simulink model "InductionHeating_bb_4"  (R2026b)
settings: Solver=FixedStepDiscrete  StopTime=0.008
PostLoadFcn:
  | Ts = 1e-6;Ts_fpga=10e-9;   R=3; Capa=300e-9;L=100e-6;Pejo_factor=1;
InitFcn:
  | Ts = 1e-6;Ts_fpga=10e-9;   R=3; Capa=300e-9;L=100e-6;Pejo_factor=1;
undefined symbols (not defined in the file or in its folder): DiscIntNeverNeededParam, ee_sli_rtmsupport, gcbh, isSetWhenUndefinedState, MATESOCwDio
libraries: fl_lib x67, nesl_utility x40, hdlsllib x32, simulink x15, eeGeneralControl x9, ee_lib x3
(part 5 of 7)

== system InductionHeating_bb_4/soc16/PWM_Generator at Ts1 ==
  note: must change deadtime because integrator reset must be scalar
  PWMsteps : Inport
  PWMstepsON : Inport  Port=2
  deatime(s) : Inport  Port=3
  enable : Inport  Port=4
  Constant : Constant  Value=[0 0]  OutDataTypeStr=boolean  SampleTime=Ts
  Data Type Conversion1 : DataTypeConversion  Commented=on  OutDataTypeStr=single  RndMeth=Nearest  SaturateOnIntegerOverflow=off
  Discrete-Time Integrator : DiscreteIntegrator  Commented=on  gainval=1  ExternalReset=level  SampleTime=Ts  LimitOutput=on  ICPrevOutput=DiscIntNeverNeededParam  ICPrevScaledInput=DiscIntNeverNeededParam
  Logical Operator1 : Logic  Operator=NOT  AllPortsSameDT=off  OutDataTypeStr=boolean
  Logical Operator2 : Logic  Commented=on  AllPortsSameDT=off  OutDataTypeStr=boolean
  Logical Operator3 : Logic  Commented=on  Operator=NOT  AllPortsSameDT=off  OutDataTypeStr=boolean
  Mux1 : Mux  Inputs=2
  PWM generator : Subsystem
  Relational Operator1 : RelationalOperator  Commented=on  Operator=>  OutDataTypeStr=boolean  RndMeth=Simplest  InputSameDT=off
  Switch : Switch  Criteria=u2 ~= 0  SaturateOnIntegerOverflow=off  InputSameDT=off
  gate : Outport  VectorParamsAs1DForOutWhenUnconnected=off
  wires:
  Constant/1 -> Switch/3
  enable/1 -> Switch/2
  Switch/1 -> gate/1
  PWMstepsON/1 -> PWM generator/2(stepON)
  PWMsteps/1 -> PWM generator/1(steps)
  PWM generator/1(pulse) -> Mux1/1, Logical Operator1/1
  Discrete-Time Integrator/1 -> Relational Operator1/1
  Relational Operator1/1 -> Logical Operator2/1
  Logical Operator3/1 -> Discrete-Time Integrator/2
  Logical Operator1/1 -> Mux1/2
  Mux1/1 -> Logical Operator2/2, Switch/1, Data Type Conversion1/1, Logical Operator3/1
  Data Type Conversion1/1 -> Discrete-Time Integrator/1  "Simulink-PS Converter1"
  deatime(s)/1 -> Relational Operator1/2

== system InductionHeating_bb_4/soc16/PWM_Generator at Ts2 ==
  note: must change deadtime because integrator reset must be scalar
  PWMsteps : Inport
  PWMstepsON : Inport  Port=2
  deatime(s) : Inport  Port=3
  enable : Inport  Port=4
  Constant : Constant  Value=[0 0]  OutDataTypeStr=boolean  SampleTime=Ts
  Data Type Conversion1 : DataTypeConversion  Commented=on  OutDataTypeStr=single  RndMeth=Nearest  SaturateOnIntegerOverflow=off
  Discrete-Time Integrator : DiscreteIntegrator  Commented=on  gainval=1  ExternalReset=level  SampleTime=Ts  LimitOutput=on  ICPrevOutput=DiscIntNeverNeededParam  ICPrevScaledInput=DiscIntNeverNeededParam
  Logical Operator1 : Logic  Operator=NOT  AllPortsSameDT=off  OutDataTypeStr=boolean
  Logical Operator2 : Logic  Commented=on  AllPortsSameDT=off  OutDataTypeStr=boolean
  Logical Operator3 : Logic  Commented=on  Operator=NOT  AllPortsSameDT=off  OutDataTypeStr=boolean
  Mux1 : Mux  Inputs=2
  PWM generator : Subsystem
  Relational Operator1 : RelationalOperator  Commented=on  Operator=>  OutDataTypeStr=boolean  RndMeth=Simplest  InputSameDT=off
  Switch : Switch  Criteria=u2 ~= 0  SaturateOnIntegerOverflow=off  InputSameDT=off
  gate : Outport  VectorParamsAs1DForOutWhenUnconnected=off
  wires:
  deatime(s)/1 -> Relational Operator1/2
  Data Type Conversion1/1 -> Discrete-Time Integrator/1  "Simulink-PS Converter1"
  Mux1/1 -> Logical Operator3/1, Data Type Conversion1/1, Switch/1, Logical Operator2/2
  Logical Operator1/1 -> Mux1/2
  Logical Operator3/1 -> Discrete-Time Integrator/2
  Relational Operator1/1 -> Logical Operator2/1
  Discrete-Time Integrator/1 -> Relational Operator1/1
  PWM generator/1(pulse) -> Logical Operator1/1, Mux1/1
  PWMsteps/1 -> PWM generator/1(steps)
  PWMstepsON/1 -> PWM generator/2(stepON)
  Switch/1 -> gate/1
  enable/1 -> Switch/2
  Constant/1 -> Switch/3

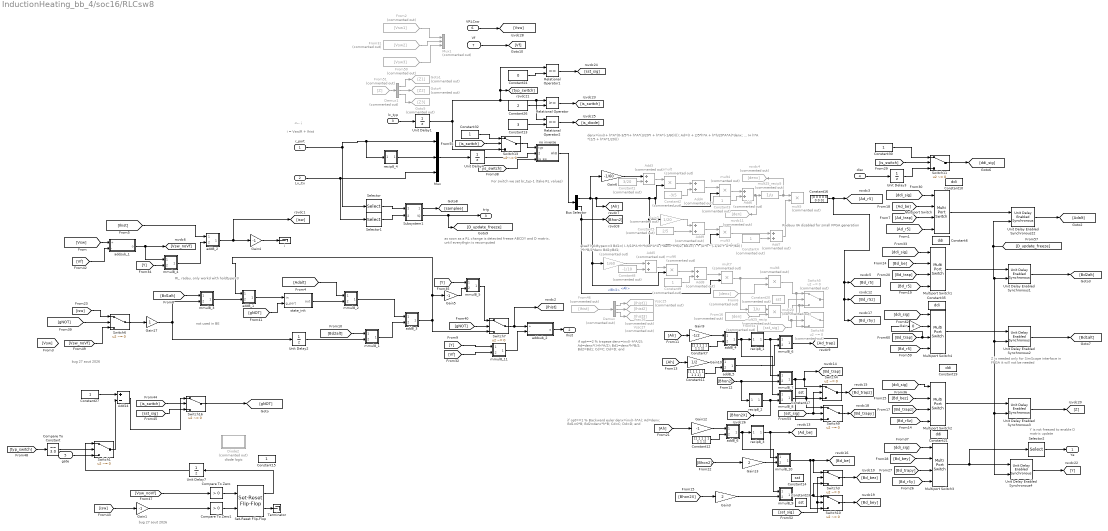
== system InductionHeating_bb_4/soc16/RLCsw8 ==
  note: Radauu IIA disabled for small FPGA generation
  note: bug 27 aout 2026
  note: bug 27 aout 2026
  note: diode logic
  note: Y is not freezed to
      | enable D matrix update
  note: as soon as a RL change is detected
      | freeze ABCDY and D matrix, until everythgin is recomputed
  note: For switch we set br_typ-1 (take RL values)
  note: if opt==1 % Backward euler
      | denx=inv(I-h*A);
      | Ad=denx;
      | Bd1=0*B;
      | Bd2=denx*h*B;
      | Cd=C;
      | Dd=D;
      | end
  note: if opt==2 % trapeze
      | denx=inv(I-h*A/2);
      | Ad=denx*(I+h*A/2);
      | Bd1=denx*h*B/2;
      | Bd2=Bd1;
      | Cd=C;
      | Dd=D;
      | end
  note: RL, radau, only workd with holdtype=3
  note: elseif holdtype==3
      | Bd1=( I-h/10*A+h*h/60*A*A )*denx*h*B/2;
      | Bd1=( I + (A*h * (-1/10 + A*h*/60) ) )*h*B/2*denx
      | Bd2=Bd1;
  note: denx=inv(I+ h*A*(0-3/5*I+ h*A*(3/20*I + h*A*(-1/60))));
      | Ad=(I + 2/5*h*A + h*h/20*A*A)*denx;
      | ... I+ h*A *(2/5 + h*A*1/20)))
  note: <-- i
  note: i = Vsw/R + Ihist
  note: Z is needed only for SimScape interface
      | in FPGA it will not be needed
  note: not used in BE
  r_port : Inport
  Lx_Cx : Inport  Port=2
  lc_typ : Inport  Port=3
  disc : Inport  Port=4
  gate : Inport  Port=5
  VRLCsw : Inport  Port=6
  Vf : Inport  Port=7
  Add14 : Sum  Inputs=+-
  Add{3..9} (7 alike) : Sum  Commented=on  Inputs=2
  Bus Selector : BusSelector  OutputSignals=Ah,Bh/2
  Compare To Constant : simulink/Logic and Bit Operations/Compare To Constant  relop===  const=3.0  OutDataTypeStr=boolean
  Compare To Zero : simulink/Logic and Bit Operations/Compare To Zero  relop=>  OutDataTypeStr=boolean
  Compare To Zero1 : simulink/Logic and Bit Operations/Compare To Zero  relop=>  OutDataTypeStr=boolean
  Constant1 : Constant  Commented=on  Value=3/20  OutDataTypeStr=single  SampleTime=Ts
  Constant{6,10,19,21,35} (5 alike) : Constant  Value=ddi  SampleTime=Ts
  Constant11 : Constant  Value=[1 1 1 1 1 1 1 1]  OutDataTypeStr=single  SampleTime=Ts
  Constant12 : Constant  Value=[1 1 1 1 1 1 1 1]  OutDataTypeStr=single  SampleTime=Ts
  Constant13 : Constant  Value=3  OutDataTypeStr=uint8  SampleTime=Ts
  Constant14 : Constant  Value=sst  SampleTime=Ts
  Constant15 : Constant  OutDataTypeStr=boolean  SampleTime=Ts
  Constant16 : Constant  Value=[0 0 0 0 0 0 0 0]  OutDataTypeStr=single  SampleTime=Ts
  Constant17 : Constant  Value=sst  SampleTime=Ts
  Constant2 : Constant  Commented=on  Value=-3/5  OutDataTypeStr=single  SampleTime=Ts
  Constant20 : Constant  Commented=on  Value=sst  SampleTime=Ts
  Constant23 : Constant  Value=sst  SampleTime=Ts
  Constant24 : Constant  Value=0  OutDataTypeStr=uint8  SampleTime=Ts
  Constant26 : Constant  Value=2  OutDataTypeStr=uint8  SampleTime=Ts
  Constant27 : Constant  OutDataTypeStr=boolean  SampleTime=Ts
  Constant3 : Constant  Commented=on  OutDataTypeStr=single  SampleTime=Ts
  Constant30 : Constant  OutDataTypeStr=uint8  SampleTime=Ts
  Constant32 : Constant  OutDataTypeStr=uint8  SampleTime=Ts
  Constant4 : Constant  Commented=on  OutDataTypeStr=single  SampleTime=Ts
  Constant5 : Constant  Commented=on  Value=2/5  OutDataTypeStr=single  SampleTime=Ts
  Constant7 : Constant  Value=[1 1 1 1 1 1 1 1]  OutDataTypeStr=single  SampleTime=Ts
  Constant8 : Constant  Commented=on  Value=-1/10  OutDataTypeStr=single  SampleTime=Ts
  Constant9 : Constant  Commented=on  OutDataTypeStr=single  SampleTime=Ts
  Demux : Demux  Commented=on  Outputs=3
  Demux1 : Demux  Commented=on  Outputs=3
  Diode2 : Subsystem  Commented=on  AncestorBlock=simetranss/FPGA/Diode  mask(MATE Diode (Pejovic-based)){VF=0.8, RON=1e-1, LON=1e-6*Pejo_factor, TS=Ts}
      mask prompts: VF "Threshold voltage (V)"; RON "Conduction resistance (Ohms)"; LON "Pejovic Equivalent Inductance during conduction (H)"; TS "Sample time (s)"
      mask help:
      | Implements a diode using a Pejovic switch model.
      |
      | Diode turns ON when Vdiode> Vthreshold and turns OFF when current is 0.
      |
      | The model is based on a Pejovic switch, with equivalent inductance during conduction Lon equal to Lon/Ts=Ts/Coff
      | where Ts is the sample time in second and Coff is the equivalent capacitance when the diode in not conducting.
  From16 : From  Commented=on  GotoTag=den
  From2 : From  Commented=on  GotoTag=Vsw1
  From31 : From  Commented=on  GotoTag=Vsw2
  From46 : From  Commented=on  GotoTag=Ihist
  From50 : From  Commented=on  GotoTag=Vsw3
  From51 : From  Commented=on  GotoTag=Z
  From54 : From  Commented=on  GotoTag=sst_sig
  From6 : From  Commented=on  GotoTag=denx
  Gain : Gain  Gain=0
  Gain{1,4..5,12} (4 alike) : Gain  Gain=-1
  Gain10 : Gain  Gain=1/2
  Gain13 : Gain  Gain=2
  Gain17 : Gain
  Gain3 : Gain  Gain=2
  Gain6 : Gain  Gain=-1/60
  Gain7 : Gain  Commented=on  Gain=1/20
  Gain8 : Gain  Commented=on  Gain=1/60
  Gain9 : Gain  Gain=-1/2
  Goto1 : Goto  Commented=on  GotoTag=Z1
  Goto4 : Goto  Commented=on  GotoTag=Z2
  Goto5 : Goto  Commented=on  GotoTag=Z3
  Multiport Switch{,1..4} (5 alike) : MultiPortSwitch  SaturateOnIntegerOverflow=off  InputSameDT=off
  Mux : Mux  Inputs=3
  Mux1 : Mux  Commented=on  Inputs=3
  Relational Operator : RelationalOperator  OutDataTypeStr=boolean  RndMeth=Simplest  InputSameDT=off
  Relational Operator1 : RelationalOperator  Operator===  OutDataTypeStr=boolean  RndMeth=Simplest  InputSameDT=off
  Relational Operator2 : RelationalOperator  Operator===  OutDataTypeStr=boolean  RndMeth=Simplest  InputSameDT=off
  Selector : Selector  InputPortWidth=8  IndexOptions=Index vector (dialog)  Indices=1  OutputSizes=1  RuntimeRangeChecks=off
  Selector1 : Selector  InputPortWidth=8  IndexOptions=Index vector (dialog)  Indices=1  OutputSizes=1  RuntimeRangeChecks=off
  Selector2 : Selector  InputPortWidth=8  IndexOptions=Index vector (dialog)  Indices=[1]  OutputSizes=1  RuntimeRangeChecks=off
  Set-Reset Flip-Flop : eeGeneralControl/Set-Reset Flip-Flop  LabelModeActiveChoice=Discrete  UndefState=Set  Q0=0  Ts=Ts
  Subsystem1 : Subsystem
  Switch1 : Switch  Criteria=u2 ~= 0  Threshold=0.5  SaturateOnIntegerOverflow=off  InputSameDT=off
  Switch{3..4,6..7,9..11} (7 alike) : Switch  Criteria=u2 ~= 0  SaturateOnIntegerOverflow=off  InputSameDT=off
  Switch13 : Switch  Criteria=u2 ~= 0  OutDataTypeStr=uint8  SaturateOnIntegerOverflow=off  InputSameDT=off
  Switch16 : Switch  Criteria=u2 ~= 0  Threshold=0.5  SaturateOnIntegerOverflow=off  InputSameDT=off
  Switch5 : Switch  Commented=on  Criteria=u2 ~= 0  SaturateOnIntegerOverflow=off  InputSameDT=off
  Switch8 : Switch  Commented=on  Criteria=u2 ~= 0  SaturateOnIntegerOverflow=off  InputSameDT=off
  Terminator : Terminator
  Unit Delay Enabled Synchronous{1..4,22} (5 alike) : hdlsllib/Discrete/Unit Delay Enabled Synchronous  InitialCondition=0.0  SampleTime=-1
  Unit Delay1 : UnitDelay  InitialCondition=1  SampleTime=Ts
  Unit Delay2 : UnitDelay  SampleTime=-1
  Unit Delay3 : UnitDelay  InitialCondition=1  SampleTime=Ts
  Unit Delay4 : UnitDelay  InitialCondition=1  SampleTime=Ts
  Unit Delay7 : UnitDelay  SampleTime=Ts
  Vssc25 : Goto  Commented=on  GotoTag=Ihist1
  Vssc26 : Goto  Commented=on  GotoTag=Ihist2
  Vssc27 : Goto  Commented=on  GotoTag=Ihist3
  add8_1 : Subsystem
      mask Display: disp('add8')
  add8_2 : Subsystem
      mask Display: disp('add8')
  add8_3 : Subsystem
      mask Display: disp('add8')
  add8_4 : Subsystem
      mask Display: disp('add8')
  add8_5 : Subsystem
      mask Display: disp('add8')
  add8_6 : Subsystem
      mask Display: disp('add8')
  addsub_1 : Subsystem
      mask Display: disp('addsub8')
  addsub_2 : Subsystem
      mask Display: disp('addsub8')
  i : Terminator
  mmul8_1 : Subsystem
      mask Display: disp('X8')
  mmul8_10 : Subsystem
      mask Display: disp('X8')
  mmul8_11 : Subsystem
      mask Display: disp('X8')
  mmul8_2 : Subsystem
      mask Display: disp('X8')
  mmul8_3 : Subsystem
      mask Display: disp('X8')
  mmul8_4 : Subsystem
      mask Display: disp('X8')
  mmul8_5 : Subsystem
      mask Display: disp('X8')
  mmul8_6 : Subsystem
      mask Display: disp('X8')
  mmul8_7 : Subsystem
      mask Display: disp('X8')
  mmul8_8 : Subsystem
      mask Display: disp('X8')
  mmul8_9 : Subsystem
      mask Display: disp('X8')
  mult{,3..8,20} (8 alike) : Product  Commented=on
  mult25_recip : Math  Commented=on  Operator=reciprocal
  mult25_recip5 : Math  Commented=on  Operator=reciprocal
  no inverse : Subsystem
  recip8_1 : Subsystem
      mask help: This block is to allow SharingFactor=8 in FPGA
      mask Display: disp('inv8')
  recip8_2 : Subsystem
      mask help: This block is to allow SharingFactor=8 in FPGA
      mask Display: disp('inv8')
  recip8_3 : Subsystem
      mask help: This block is to allow SharingFactor=8 in FPGA
      mask Display: disp('inv8')
  recip8_4 : Subsystem
      mask help: This block is to allow SharingFactor=8 in FPGA
      mask Display: disp('inv8')
  rsvdc11 : Goto  Commented=on  GotoTag=den
  rsvdc4 : Goto  Commented=on  GotoTag=denx
  state_init : Subsystem
  Ye : Outport
  Ihist : Outport  Port=2
  trig : Outport  Port=3
  wires:
  Switch16/1 -> [gNOT]
  Add14/1 -> Switch16/1
  [gNOT] -> state_init/2(g_port)
  state_init/1(out) -> mmul8_2/2(In2)
  [gNOT] -> Switch7/2
  [gNOT] -> Switch6/2
  Constant27/1 -> Add14/1
  Gain17/1 -> mmul8_3/2(In2), Unit Delay2/1
  Gain5/1 -> mmul8_5/2(In2)
  [Y] -> mmul8_5/1(In1)
  mmul8_5/1(Out1) -> Switch7/1
  mmul8_4/1(Out1) -> add8_2/2(In2)
  [Y] -> mmul8_4/2(In2)
  Switch10/1 -> [Bd_bey]
  mmul8_7/1(Out1) -> Switch4/1, [Bd_trap], Switch9/3
  mmul8_8/1(Out1) -> Switch4/3, Switch9/1
  Switch9/1 -> [Bd_trapy]
  [Bd_r5y] -> Multiport Switch3/4
  [Bd_trapy] -> Multiport Switch3/3
  [Bd_bey] -> Multiport Switch3/2
  Switch4/1 -> [Bd_trapz]
  mult8/1 -> Switch5/1, Switch8/3
  [Bd_bez] -> Multiport Switch2/2
  [Bd_trapz] -> Multiport Switch2/3
  [Bd_r5z] -> Multiport Switch2/4
  mmul8_2/1(Out1) -> add8_3/1(In1)
  [isw] -> Switch6/1
  Switch6/1 -> Gain17/1
  add8_2/1(Out1) -> [isw], Gain4/1
  [Ihist] -> add8_2/1(In1)
  Gain4/1 -> i/1
  add8_1/1(Out1) -> state_init/1(in)
  add8_3/1(Out1) -> add8_1/1(In1), Gain5/1, Switch7/3
  Gain6/1 -> Add3/1
  Constant1/1 -> Add3/2
  mult/1 -> Add4/1
  Add3/1 -> mult/1
  Constant2/1 -> Add4/2
  Add4/1 -> mult4/1
  mult4/1 -> Add6/1
  Constant3/1 -> Add6/2
  Add6/1 -> rsvdc11/1, mult25_recip5/1
  Constant4/1 -> Add7/2
  Constant5/1 -> Add9/2
  Add9/1 -> mult3/1
  Gain7/1 -> Add9/1
  mult3/1 -> Add7/1
  Add7/1 -> mult5/2
  [Adalt] -> mmul8_2/1(In1)
  mult25_recip5/1 -> rsvdc4/1, mult5/1
  Constant9/1 -> Add8/2
  Add5/1 -> mult6/1
  mult6/1 -> Add8/1
  Constant8/1 -> Add5/2
  Gain8/1 -> Add5/1
  Add8/1 -> mult7/1
  mult7/1 -> mult25_recip/1, mult8/1
  From6/1 -> mult8/2
  Bus Selector/1 -> Gain6/1, [Ah], mult3/2, Gain7/1, mult4/2, mult/2, Gain8/1, mult6/2  "<Ah>"
  Bus Selector/2 -> mult7/2, [Bhon2]  "<Bh/2>"
  [Ah] -> Gain9/1
  Gain9/1 -> add8_4/1(In1)
  Constant7/1 -> add8_4/2(In2)
  add8_4/1(Out1) -> recip8_1/1(In1), mmul8_8/1(In1)
  add8_5/1(Out1) -> mmul8_6/2(In2)
  Constant11/1 -> add8_5/2(In2)
  Gain10/1 -> add8_5/1(In1)
  [Ah] -> Gain10/1
  recip8_1/1(Out1) -> mmul8_7/1(In1), mmul8_6/1(In1)
  [Bhon2] -> recip8_2/1(In1), mmul8_7/2(In2)
  mmul8_6/1(Out1) -> [Ad_trap]
  mmul8_3/1(Out1) -> add8_1/2(In2)
  recip8_3/1(Out1) -> mmul8_10/1(In1), [Ad_be]
  [Bhon2] -> Gain13/1
  add8_6/1(Out1) -> recip8_3/1(In1), mmul8_9/1(In1)
  Constant12/1 -> add8_6/2(In2)
  Gain12/1 -> add8_6/1(In1)
  [Ah] -> Gain12/1
  Gain13/1 -> mmul8_10/2(In2)
  [Ad_r5] -> Multiport Switch/4
  [Ad_trap] -> Multiport Switch/3
  [Ad_be] -> Multiport Switch/2
  [Bd_r5] -> Multiport Switch1/4
  [Bd_trap] -> Multiport Switch1/3
  [Bd_be] -> Multiport Switch1/2
  recip8_2/1(Out1) -> [Bhon2X], mmul8_8/2(In2)
  Gain3/1 -> mmul8_9/2(In2)
  mmul8_9/1(Out1) -> Switch3/3, Switch10/1
  mmul8_10/1(Out1) -> Switch3/1, [Bd_be], Switch10/3
  Switch3/1 -> [Bd_bez]
  From16/1 -> mult20/2
  mult25_recip/1 -> mult20/1
  mult20/1 -> Switch5/3, Switch8/1
  Mux/1 -> Unit Delay4/1
  lc_typ/1 -> Unit Delay1/1
  no inverse/1(AhB) -> Bus Selector/1
  Constant26/1 -> Relational Operator/2
  Relational Operator/1 -> [is_switch]
  [is_switch] -> Switch16/2
  Constant24/1 -> Relational Operator1/2
  Relational Operator1/1 -> [sst_sig]
  [sst_sig] -> Switch16/3
  From46/1 -> Demux/1
  Demux/1 -> Vssc25/1
  Demux/2 -> Vssc26/1
  Demux/3 -> Vssc27/1
  From31/1 -> Mux1/2
  From2/1 -> Mux1/1
  From50/1 -> Mux1/3
  From51/1 -> Demux1/1
  Demux1/2 -> Goto4/1
  Demux1/1 -> Goto1/1
  Demux1/3 -> Goto5/1
  [is_switch] -> Switch11/2
  disc/1 -> Unit Delay3/1
  Constant30/1 -> Switch11/1
  Switch11/1 -> [ddi_sig]
  [ddi_sig] -> Multiport Switch/1
  [ddi_sig] -> Multiport Switch1/1
  [ddi_sig] -> Multiport Switch2/1
  [ddi_sig] -> Multiport Switch3/1
  [sst_sig] -> Switch3/2, Switch10/2
  [sst_sig] -> Switch4/2, Switch9/2
  From54/1 -> Switch8/2, Switch5/2
  r_port/1 -> recip8_4/1(In1), Mux/1, Selector/1
  ? -> ?
  Switch13/1 -> no inverse/1(typ)
  Constant32/1 -> Switch13/1
  mmul8_1/1(Out1) -> add8_3/2(In2)
  Unit Delay2/1 -> mmul8_1/2(In2)
  [ddi_sig] -> Multiport Switch4/1
  [Bd_r5] -> Multiport Switch4/4
  [Bd_trap] -> Gain/1, Multiport Switch4/3
  Lx_Cx/1 -> Mux/3, Selector1/1
  [Bd2alt] -> mmul8_1/1(In1)
  [Bd1alt] -> mmul8_3/1(In1)
  VRLCsw/1 -> [Vsw]
  Multiport Switch1/1 -> Unit Delay Enabled Synchronous1/1
  Unit Delay Enabled Synchronous22/1 -> [Adalt]
  Multiport Switch/1 -> Unit Delay Enabled Synchronous22/1
  Unit Delay Enabled Synchronous1/1 -> [Bd2alt]
  Multiport Switch4/1 -> Unit Delay Enabled Synchronous2/1
  Unit Delay Enabled Synchronous2/1 -> [Bd1alt]
  Multiport Switch2/1 -> Unit Delay Enabled Synchronous3/1
  Unit Delay Enabled Synchronous3/1 -> [Z]
  Multiport Switch3/1 -> Unit Delay Enabled Synchronous4/1, Selector2/1
  Unit Delay Enabled Synchronous4/1 -> [Y]
  Subsystem1/1(q_port) -> [samplee]
  Selector/1 -> Subsystem1/1(trig)
  Selector1/1 -> Subsystem1/2(trig1)
  Subsystem1/2(!Q) -> [D_update_freeze], trig/1
  [D_update_freeze] -> Unit Delay Enabled Synchronous22/2, Unit Delay Enabled Synchronous2/2, Unit Delay Enabled Synchronous4/2, Unit Delay Enabled Synchronous3/2, Unit Delay Enabled Synchronous1/2
  Selector2/1 -> Ye/1
  Gain/1 -> Multiport Switch4/2
  [is_switch] -> Switch13/2
  Unit Delay4/1 -> no inverse/2(R_Rx_Lx_Cx)
  Unit Delay1/1 -> Relational Operator2/1, Relational Operator/1, Relational Operator1/1, [typ_switch], Switch13/3
  Unit Delay3/1 -> Switch11/3
  Switch7/1 -> [Ihist], addsub_2/1(+)
  addsub_2/1(o) -> Ihist/1
  [Y] -> mmul8_11/1(In1)
  mmul8_11/1(Out1) -> addsub_2/2(-)
  [Vsw] -> addsub_1/1(+)
  addsub_1/1(o) -> mmul8_4/1(In1), [Vsw_noVf]
  [Vf] -> mmul8_11/2(In2)
  Vf/1 -> [Vf]
  [Vf] -> addsub_1/2(-)
  Set-Reset Flip-Flop/2 -> Terminator/1
  [isw] -> Gain1/1
  Compare To Zero/1 -> Set-Reset Flip-Flop/1
  [Vsw_noVf] -> Compare To Zero/1
  Compare To Zero1/1 -> Set-Reset Flip-Flop/2
  Unit Delay7/1 -> Switch1/1
  [typ_switch] -> Compare To Constant/1
  gate/1 -> Switch1/3
  Switch1/1 -> Add14/2
  Compare To Constant/1 -> Switch1/2
  Constant13/1 -> Relational Operator2/2
  Relational Operator2/1 -> [is_diode]
  recip8_4/1(Out1) -> Mux/2
  [is_switch] -> no inverse/3(is_sw)
  Gain1/1 -> Compare To Zero1/1
  [Vsw_noVf] -> Switch6/3
  Set-Reset Flip-Flop/1 -> Unit Delay7/1
  Constant16/1 -> [Bd_r5y], [Bd_r5z], [Bd_r5], [Ad_r5]
  [Bhon2X] -> Gain3/1

== system InductionHeating_bb_4/MATEwDiode/C1/RC.1 ==
  RLC : Inport
  typ : Inport  Port=2
  Bus Creator : BusCreator  Inputs=2
  Demux : Demux  Outputs=2
  Divide : Product  Inputs=*/
  Divide1 : Product  Inputs=/
  Divide3 : Product
  Divide4 : Product  Inputs=/
  Divide5 : Product  Inputs=/
  Gain : Gain  Gain=-Ts
  Gain1 : Gain  Gain=Ts/2
  Gain2 : Gain  Gain=Ts/2
  Gain3 : Gain  Gain=-Ts
  Switch : Switch  Criteria=u2 > Threshold  SaturateOnIntegerOverflow=off  InputSameDT=off
  Switch1 : Switch  Criteria=u2 > Threshold  SaturateOnIntegerOverflow=off  InputSameDT=off
  AhB : Outport
  wires:
  Gain2/1 -> Switch1/1  "Bh/2"
  Gain3/1 -> Switch/1  "Ah"
  Gain1/1 -> Switch1/3  "Bh/2"
  Gain/1 -> Switch/3  "Ah"
  typ/1 -> Switch/2, Switch1/2
  Switch1/1 -> Bus Creator/2  "Bh/2"
  Switch/1 -> Bus Creator/1  "Ah"
  Divide3/1 -> Gain3/1
  Divide4/1 -> Divide3/2, Gain2/1
  RLC/1 -> Demux/1
  Bus Creator/1 -> AhB/1
  Demux/1 -> Divide5/1, Divide/1
  Divide1/1 -> Gain1/1
  Divide/1 -> Gain/1
  Demux/2 -> Divide1/1, Divide/2, Divide4/1
  Divide5/1 -> Divide3/1

== system InductionHeating_bb_4/MATEwDiode/C1/Rsw ==
  Variable Resistor : fl_lib/Electrical/Electrical Elements/Variable Resistor  Rmin=1e-8 Ohm  thermalEnable=false  thermal_mass=1 J/K  i_specify=off  i_priority=None  i=0 A  i_nominal_specify=off  i_nominal_value=1  i_nominal_unit=A  v_specify=off  v_priority=None  v=0 V  v_nominal_specify=off  v_nominal_value=1  v_nominal_unit=V  T_specify=off  T_priority=None  T=300 K  T_nominal_specify=off  T_nominal_value=1  T_nominal_unit=K
  + : PMIOPort  Side=Left
  R : PMIOPort  Port=2  Side=Left
  - : PMIOPort  Port=3  Side=Right
  connections:
  Variable Resistor/RConn1 -- -/RConn1
  Variable Resistor/LConn2 -- +/RConn1
  R/RConn1 -- Variable Resistor/LConn1

== system InductionHeating_bb_4/MATEwDiode/C1/state_init ==
  in : Inport
  g : Inport  Port=2
  Gain18 : Gain
  Relational Operator1 : RelationalOperator  Operator=~=  OutDataTypeStr=boolean  RndMeth=Simplest  InputSameDT=off
  Switch16 : Switch  Criteria=u2 ~= 0  Threshold=0.5  SaturateOnIntegerOverflow=off  InputSameDT=off
  Unit Delay6 : UnitDelay  SampleTime=-1
  Unit Delay7 : UnitDelay  SampleTime=Ts
  Unit Delay8 : UnitDelay  SampleTime=Ts
  init_in : Constant  Value=0
  out : Outport
  wires:
  Unit Delay8/1 -> Relational Operator1/1
  Relational Operator1/1 -> Gain18/1
  Unit Delay6/1 -> Switch16/3
  init_in/1 -> Unit Delay7/1
  Gain18/1 -> Switch16/2
  Unit Delay7/1 -> Switch16/1
  in/1 -> Unit Delay6/1
  Switch16/1 -> out/1
  g/1 -> Unit Delay8/1, Relational Operator1/2

== system InductionHeating_bb_4/MATEwDiode/C2/RC.1 ==
  RLC : Inport
  typ : Inport  Port=2
  Bus Creator : BusCreator  Inputs=2
  Demux : Demux  Outputs=2
  Divide : Product  Inputs=*/
  Divide1 : Product  Inputs=/
  Divide3 : Product
  Divide4 : Product  Inputs=/
  Divide5 : Product  Inputs=/
  Gain : Gain  Gain=-Ts
  Gain1 : Gain  Gain=Ts/2
  Gain2 : Gain  Gain=Ts/2
  Gain3 : Gain  Gain=-Ts
  Switch : Switch  Criteria=u2 > Threshold  SaturateOnIntegerOverflow=off  InputSameDT=off
  Switch1 : Switch  Criteria=u2 > Threshold  SaturateOnIntegerOverflow=off  InputSameDT=off
  AhB : Outport
  wires:
  Gain2/1 -> Switch1/1  "Bh/2"
  Gain3/1 -> Switch/1  "Ah"
  Gain1/1 -> Switch1/3  "Bh/2"
  Gain/1 -> Switch/3  "Ah"
  typ/1 -> Switch/2, Switch1/2
  Switch1/1 -> Bus Creator/2  "Bh/2"
  Switch/1 -> Bus Creator/1  "Ah"
  Divide3/1 -> Gain3/1
  Divide4/1 -> Divide3/2, Gain2/1
  RLC/1 -> Demux/1
  Bus Creator/1 -> AhB/1
  Demux/1 -> Divide5/1, Divide/1
  Divide1/1 -> Gain1/1
  Divide/1 -> Gain/1
  Demux/2 -> Divide1/1, Divide/2, Divide4/1
  Divide5/1 -> Divide3/1

== system InductionHeating_bb_4/MATEwDiode/C2/Rsw ==
  Variable Resistor : fl_lib/Electrical/Electrical Elements/Variable Resistor  Rmin=1e-8 Ohm  thermalEnable=false  thermal_mass=1 J/K  i_specify=off  i_priority=None  i=0 A  i_nominal_specify=off  i_nominal_value=1  i_nominal_unit=A  v_specify=off  v_priority=None  v=0 V  v_nominal_specify=off  v_nominal_value=1  v_nominal_unit=V  T_specify=off  T_priority=None  T=300 K  T_nominal_specify=off  T_nominal_value=1  T_nominal_unit=K
  + : PMIOPort  Side=Left
  R : PMIOPort  Port=2  Side=Left
  - : PMIOPort  Port=3  Side=Right
  connections:
  Variable Resistor/RConn1 -- -/RConn1
  Variable Resistor/LConn2 -- +/RConn1
  R/RConn1 -- Variable Resistor/LConn1

== system InductionHeating_bb_4/MATEwDiode/C2/state_init ==
  in : Inport
  g : Inport  Port=2
  Gain18 : Gain
  Relational Operator1 : RelationalOperator  Operator=~=  OutDataTypeStr=boolean  RndMeth=Simplest  InputSameDT=off
  Switch16 : Switch  Criteria=u2 ~= 0  Threshold=0.5  SaturateOnIntegerOverflow=off  InputSameDT=off
  Unit Delay6 : UnitDelay  SampleTime=-1
  Unit Delay7 : UnitDelay  SampleTime=Ts
  Unit Delay8 : UnitDelay  SampleTime=Ts
  init_in : Constant  Value=0
  out : Outport
  wires:
  Unit Delay8/1 -> Relational Operator1/1
  Relational Operator1/1 -> Gain18/1
  Unit Delay6/1 -> Switch16/3
  init_in/1 -> Unit Delay7/1
  Gain18/1 -> Switch16/2
  Unit Delay7/1 -> Switch16/1
  in/1 -> Unit Delay6/1
  Switch16/1 -> out/1
  g/1 -> Unit Delay8/1, Relational Operator1/2

== system InductionHeating_bb_4/MATEwDiode/Cdc/RC.1 ==
  RLC : Inport
  typ : Inport  Port=2
  Bus Creator : BusCreator  Inputs=2
  Demux : Demux  Outputs=2
  Divide : Product  Inputs=*/
  Divide1 : Product  Inputs=/
  Divide3 : Product
  Divide4 : Product  Inputs=/
  Divide5 : Product  Inputs=/
  Gain : Gain  Gain=-Ts
  Gain1 : Gain  Gain=Ts/2
  Gain2 : Gain  Gain=Ts/2
  Gain3 : Gain  Gain=-Ts
  Switch : Switch  Criteria=u2 > Threshold  SaturateOnIntegerOverflow=off  InputSameDT=off
  Switch1 : Switch  Criteria=u2 > Threshold  SaturateOnIntegerOverflow=off  InputSameDT=off
  AhB : Outport
  wires:
  Divide5/1 -> Divide3/1
  Demux/2 -> Divide4/1, Divide/2, Divide1/1
  Divide/1 -> Gain/1
  Divide1/1 -> Gain1/1
  Demux/1 -> Divide/1, Divide5/1
  Bus Creator/1 -> AhB/1
  RLC/1 -> Demux/1
  Divide4/1 -> Gain2/1, Divide3/2
  Divide3/1 -> Gain3/1
  Switch/1 -> Bus Creator/1  "Ah"
  Switch1/1 -> Bus Creator/2  "Bh/2"
  typ/1 -> Switch1/2, Switch/2
  Gain/1 -> Switch/3  "Ah"
  Gain1/1 -> Switch1/3  "Bh/2"
  Gain3/1 -> Switch/1  "Ah"
  Gain2/1 -> Switch1/1  "Bh/2"

== system InductionHeating_bb_4/MATEwDiode/Cdc/Rsw ==
  Variable Resistor : fl_lib/Electrical/Electrical Elements/Variable Resistor  Rmin=1e-8 Ohm  thermalEnable=false  thermal_mass=1 J/K  i_specify=off  i_priority=None  i=0 A  i_nominal_specify=off  i_nominal_value=1  i_nominal_unit=A  v_specify=off  v_priority=None  v=0 V  v_nominal_specify=off  v_nominal_value=1  v_nominal_unit=V  T_specify=off  T_priority=None  T=300 K  T_nominal_specify=off  T_nominal_value=1  T_nominal_unit=K
  + : PMIOPort  Side=Left
  R : PMIOPort  Port=2  Side=Left
  - : PMIOPort  Port=3  Side=Right
  connections:
  R/RConn1 -- Variable Resistor/LConn1
  Variable Resistor/LConn2 -- +/RConn1
  Variable Resistor/RConn1 -- -/RConn1

== system InductionHeating_bb_4/MATEwDiode/Cdc/state_init ==
  in : Inport
  g : Inport  Port=2
  Gain18 : Gain
  Relational Operator1 : RelationalOperator  Operator=~=  OutDataTypeStr=boolean  RndMeth=Simplest  InputSameDT=off
  Switch16 : Switch  Criteria=u2 ~= 0  Threshold=0.5  SaturateOnIntegerOverflow=off  InputSameDT=off
  Unit Delay6 : UnitDelay  SampleTime=-1
  Unit Delay7 : UnitDelay  SampleTime=Ts
  Unit Delay8 : UnitDelay  SampleTime=Ts
  init_in : Constant  Value=0
  out : Outport
  wires:
  g/1 -> Relational Operator1/2, Unit Delay8/1
  Switch16/1 -> out/1
  in/1 -> Unit Delay6/1
  Unit Delay7/1 -> Switch16/1
  Gain18/1 -> Switch16/2
  init_in/1 -> Unit Delay7/1
  Unit Delay6/1 -> Switch16/3
  Relational Operator1/1 -> Gain18/1
  Unit Delay8/1 -> Relational Operator1/1

== system InductionHeating_bb_4/MATEwDiode/Diode1/Pejovic L-C-switch component ==
  gate : Inport
  Vf : Inport  Port=2
  Add : Sum  Inputs=+-
  Add1 : Sum  Inputs=2
  Add2 : Sum  Inputs=+-
  Add3 : Sum  Inputs=2
  Add4 : Sum  Inputs=+-
  CCS1 : fl_lib/Electrical/Electrical Sources/Controlled Current Source
  Gain1 : Gain  Gain=-1/Rsw
  Gain2 : Gain  Gain=Xcomp
  Gain3 : Gain  Gain=-1
  Gain4 : Gain  Gain=-1
  Gain5 : Gain  Gain=1/Rsw*traprule
  Gain6 : Gain  Gain=traprule
  Gain7 : Gain  Gain=-1/Rsw
  PS-Simulink Converter2 : nesl_utility/PS-Simulink Converter  PhysicalDomain=network_engine_domain  SubClassName=ps_output  LeftPortType=input  RightPortType=output  PseudoPeriodic=off  Frequencies=[]  VectorFormat=inherit  Unit=inherit  AffineConversion=off
  Relational Operator1 : RelationalOperator  Operator=~=  OutDataTypeStr=boolean  RndMeth=Simplest  InputSameDT=off
  Resistor : fl_lib/Electrical/Electrical Elements/Resistor  R=Rsw Ohm  i_specify=off  i_priority=None  i=0 A  i_nominal_specify=off  i_nominal_value=1  i_nominal_unit=A  v_specify=off  v_priority=None  v=0 V  v_nominal_specify=off  v_nominal_value=1  v_nominal_unit=V
  Simulink-PS Converter1 : nesl_utility/Simulink-PS Converter  PhysicalDomain=network_engine_domain  SubClassName=ps_input  LeftPortType=input  RightPortType=output  PseudoPeriodic=off  Frequencies=[]  NoiseDistribution=none  NoiseParameters=[]  Unit=1  AffineConversion=off  FilteringAndDerivatives=provide  SimscapeFilterOrder=1  InputFilterTimeConstant=0.001  UdotUserProvided=0
  Switch : Switch  Criteria=u2 > Threshold  Threshold=0.5  SaturateOnIntegerOverflow=off  InputSameDT=off
  Switch4 : Switch  Criteria=u2 > Threshold  Threshold=0.5  SaturateOnIntegerOverflow=off  InputSameDT=off
  Switch5 : Switch  Criteria=u2 ~= 0  Threshold=0.5  SaturateOnIntegerOverflow=off  InputSameDT=off
  Unit Delay1 : UnitDelay  SampleTime=-1
  Unit Delay2 : UnitDelay  SampleTime=Ts
  Unit Delay6 : UnitDelay  SampleTime=Ts
  VS1 : fl_lib/Electrical/Electrical Sensors/Voltage Sensor
  init_in : Constant
  init_out : Terminator
  +V : PMIOPort  Side=Left
  -V : PMIOPort  Port=2  Side=Right
  v : Outport
  i : Outport  Port=2
  wires:
  Add4/1 -> [Vsw], v/1
  Add3/1 -> Simulink-PS Converter1/1
  Gain7/1 -> Add3/2
  [Ihist] -> Add3/1
  Vf/1 -> Gain7/1, Add4/2
  Gain6/1 -> Add2/2
  Add2/1 -> Switch/3
  Gain5/1 -> Add1/2
  [Vsw] -> Gain5/1
  Add1/1 -> Switch/1
  Gain4/1 -> i/1
  Switch5/1 -> [Ihist]
  init_in/1 -> Unit Delay2/1
  Relational Operator1/1 -> Gain2/1
  gate/1 -> Switch/2, Relational Operator1/2, Unit Delay6/1, Switch4/2
  Unit Delay6/1 -> Relational Operator1/1
  Gain2/1 -> Switch5/2
  Gain3/1 -> Switch4/1
  Switch4/1 -> init_out/1
  Unit Delay1/1 -> Switch5/3
  Gain1/1 -> Add/2, Add2/1
  [Ihist] -> Add/1
  PS-Simulink Converter2/1 -> Add4/1
  [Vsw] -> Gain1/1
  Switch/1 -> Unit Delay1/1
  Add/1 -> Gain4/1, Add1/1, Gain6/1
  [Ihist] -> Switch4/3, Gain3/1
  Unit Delay2/1 -> Switch5/1
  connections:
  Resistor/RConn1 -- CCS1/LConn1 -- VS1/RConn2 -- -V/RConn1
  PS-Simulink Converter2/LConn1 -- VS1/RConn1
  CCS1/RConn1 -- Simulink-PS Converter1/RConn1
  Resistor/LConn1 -- VS1/LConn1 -- +V/RConn1 -- CCS1/RConn2

== system InductionHeating_bb_4/MATEwDiode/Diode2/Pejovic L-C-switch component ==
  gate : Inport
  Vf : Inport  Port=2
  Add : Sum  Inputs=+-
  Add1 : Sum  Inputs=2
  Add2 : Sum  Inputs=+-
  Add3 : Sum  Inputs=2
  Add4 : Sum  Inputs=+-
  CCS1 : fl_lib/Electrical/Electrical Sources/Controlled Current Source
  Gain1 : Gain  Gain=-1/Rsw
  Gain2 : Gain  Gain=Xcomp
  Gain3 : Gain  Gain=-1
  Gain4 : Gain  Gain=-1
  Gain5 : Gain  Gain=1/Rsw*traprule
  Gain6 : Gain  Gain=traprule
  Gain7 : Gain  Gain=-1/Rsw
  PS-Simulink Converter2 : nesl_utility/PS-Simulink Converter  PhysicalDomain=network_engine_domain  SubClassName=ps_output  LeftPortType=input  RightPortType=output  PseudoPeriodic=off  Frequencies=[]  VectorFormat=inherit  Unit=inherit  AffineConversion=off
  Relational Operator1 : RelationalOperator  Operator=~=  OutDataTypeStr=boolean  RndMeth=Simplest  InputSameDT=off
  Resistor : fl_lib/Electrical/Electrical Elements/Resistor  R=Rsw Ohm  i_specify=off  i_priority=None  i=0 A  i_nominal_specify=off  i_nominal_value=1  i_nominal_unit=A  v_specify=off  v_priority=None  v=0 V  v_nominal_specify=off  v_nominal_value=1  v_nominal_unit=V
  Simulink-PS Converter1 : nesl_utility/Simulink-PS Converter  PhysicalDomain=network_engine_domain  SubClassName=ps_input  LeftPortType=input  RightPortType=output  PseudoPeriodic=off  Frequencies=[]  NoiseDistribution=none  NoiseParameters=[]  Unit=1  AffineConversion=off  FilteringAndDerivatives=provide  SimscapeFilterOrder=1  InputFilterTimeConstant=0.001  UdotUserProvided=0
  Switch : Switch  Criteria=u2 > Threshold  Threshold=0.5  SaturateOnIntegerOverflow=off  InputSameDT=off
  Switch4 : Switch  Criteria=u2 > Threshold  Threshold=0.5  SaturateOnIntegerOverflow=off  InputSameDT=off
  Switch5 : Switch  Criteria=u2 ~= 0  Threshold=0.5  SaturateOnIntegerOverflow=off  InputSameDT=off
  Unit Delay1 : UnitDelay  SampleTime=-1
  Unit Delay2 : UnitDelay  SampleTime=Ts
  Unit Delay6 : UnitDelay  SampleTime=Ts
  VS1 : fl_lib/Electrical/Electrical Sensors/Voltage Sensor
  init_in : Constant
  init_out : Terminator
  +V : PMIOPort  Side=Left
  -V : PMIOPort  Port=2  Side=Right
  v : Outport
  i : Outport  Port=2
  wires:
  Unit Delay2/1 -> Switch5/1
  [Ihist] -> Gain3/1, Switch4/3
  Add/1 -> Gain6/1, Add1/1, Gain4/1
  Switch/1 -> Unit Delay1/1
  [Vsw] -> Gain1/1
  PS-Simulink Converter2/1 -> Add4/1
  [Ihist] -> Add/1
  Gain1/1 -> Add2/1, Add/2
  Unit Delay1/1 -> Switch5/3
  Switch4/1 -> init_out/1
  Gain3/1 -> Switch4/1
  Gain2/1 -> Switch5/2
  Unit Delay6/1 -> Relational Operator1/1
  gate/1 -> Switch4/2, Unit Delay6/1, Relational Operator1/2, Switch/2
  Relational Operator1/1 -> Gain2/1
  init_in/1 -> Unit Delay2/1
  Switch5/1 -> [Ihist]
  Gain4/1 -> i/1
  Add1/1 -> Switch/1
  [Vsw] -> Gain5/1
  Gain5/1 -> Add1/2
  Add2/1 -> Switch/3
  Gain6/1 -> Add2/2
  Vf/1 -> Add4/2, Gain7/1
  [Ihist] -> Add3/1
  Gain7/1 -> Add3/2
  Add3/1 -> Simulink-PS Converter1/1
  Add4/1 -> v/1, [Vsw]
  connections:
  CCS1/RConn2 -- +V/RConn1 -- VS1/LConn1 -- Resistor/LConn1
  CCS1/RConn1 -- Simulink-PS Converter1/RConn1
  PS-Simulink Converter2/LConn1 -- VS1/RConn1
  -V/RConn1 -- VS1/RConn2 -- CCS1/LConn1 -- Resistor/RConn1

== system InductionHeating_bb_4/MATEwDiode/Diode3/Pejovic L-C-switch component ==
  gate : Inport
  Vf : Inport  Port=2
  Add : Sum  Inputs=+-
  Add1 : Sum  Inputs=2
  Add2 : Sum  Inputs=+-
  Add3 : Sum  Inputs=2
  Add4 : Sum  Inputs=+-
  CCS1 : fl_lib/Electrical/Electrical Sources/Controlled Current Source
  Gain1 : Gain  Gain=-1/Rsw
  Gain2 : Gain  Gain=Xcomp
  Gain3 : Gain  Gain=-1
  Gain4 : Gain  Gain=-1
  Gain5 : Gain  Gain=1/Rsw*traprule
  Gain6 : Gain  Gain=traprule
  Gain7 : Gain  Gain=-1/Rsw
  PS-Simulink Converter2 : nesl_utility/PS-Simulink Converter  PhysicalDomain=network_engine_domain  SubClassName=ps_output  LeftPortType=input  RightPortType=output  PseudoPeriodic=off  Frequencies=[]  VectorFormat=inherit  Unit=inherit  AffineConversion=off
  Relational Operator1 : RelationalOperator  Operator=~=  OutDataTypeStr=boolean  RndMeth=Simplest  InputSameDT=off
  Resistor : fl_lib/Electrical/Electrical Elements/Resistor  R=Rsw Ohm  i_specify=off  i_priority=None  i=0 A  i_nominal_specify=off  i_nominal_value=1  i_nominal_unit=A  v_specify=off  v_priority=None  v=0 V  v_nominal_specify=off  v_nominal_value=1  v_nominal_unit=V
  Simulink-PS Converter1 : nesl_utility/Simulink-PS Converter  PhysicalDomain=network_engine_domain  SubClassName=ps_input  LeftPortType=input  RightPortType=output  PseudoPeriodic=off  Frequencies=[]  NoiseDistribution=none  NoiseParameters=[]  Unit=1  AffineConversion=off  FilteringAndDerivatives=provide  SimscapeFilterOrder=1  InputFilterTimeConstant=0.001  UdotUserProvided=0
  Switch : Switch  Criteria=u2 > Threshold  Threshold=0.5  SaturateOnIntegerOverflow=off  InputSameDT=off
  Switch4 : Switch  Criteria=u2 > Threshold  Threshold=0.5  SaturateOnIntegerOverflow=off  InputSameDT=off
  Switch5 : Switch  Criteria=u2 ~= 0  Threshold=0.5  SaturateOnIntegerOverflow=off  InputSameDT=off
  Unit Delay1 : UnitDelay  SampleTime=-1
  Unit Delay2 : UnitDelay  SampleTime=Ts
  Unit Delay6 : UnitDelay  SampleTime=Ts
  VS1 : fl_lib/Electrical/Electrical Sensors/Voltage Sensor
  init_in : Constant
  init_out : Terminator
  +V : PMIOPort  Side=Left
  -V : PMIOPort  Port=2  Side=Right
  v : Outport
  i : Outport  Port=2
  wires:
  Unit Delay2/1 -> Switch5/1
  [Ihist] -> Gain3/1, Switch4/3
  Add/1 -> Gain6/1, Add1/1, Gain4/1
  Switch/1 -> Unit Delay1/1
  [Vsw] -> Gain1/1
  PS-Simulink Converter2/1 -> Add4/1
  [Ihist] -> Add/1
  Gain1/1 -> Add2/1, Add/2
  Unit Delay1/1 -> Switch5/3
  Switch4/1 -> init_out/1
  Gain3/1 -> Switch4/1
  Gain2/1 -> Switch5/2
  Unit Delay6/1 -> Relational Operator1/1
  gate/1 -> Switch4/2, Unit Delay6/1, Relational Operator1/2, Switch/2
  Relational Operator1/1 -> Gain2/1
  init_in/1 -> Unit Delay2/1
  Switch5/1 -> [Ihist]
  Gain4/1 -> i/1
  Add1/1 -> Switch/1
  [Vsw] -> Gain5/1
  Gain5/1 -> Add1/2
  Add2/1 -> Switch/3
  Gain6/1 -> Add2/2
  Vf/1 -> Add4/2, Gain7/1
  [Ihist] -> Add3/1
  Gain7/1 -> Add3/2
  Add3/1 -> Simulink-PS Converter1/1
  Add4/1 -> v/1, [Vsw]
  connections:
  CCS1/RConn2 -- +V/RConn1 -- VS1/LConn1 -- Resistor/LConn1
  CCS1/RConn1 -- Simulink-PS Converter1/RConn1
  PS-Simulink Converter2/LConn1 -- VS1/RConn1
  -V/RConn1 -- VS1/RConn2 -- CCS1/LConn1 -- Resistor/RConn1

== system InductionHeating_bb_4/MATEwDiode/Diode4/Pejovic L-C-switch component ==
  gate : Inport
  Vf : Inport  Port=2
  Add : Sum  Inputs=+-
  Add1 : Sum  Inputs=2
  Add2 : Sum  Inputs=+-
  Add3 : Sum  Inputs=2
  Add4 : Sum  Inputs=+-
  CCS1 : fl_lib/Electrical/Electrical Sources/Controlled Current Source
  Gain1 : Gain  Gain=-1/Rsw
  Gain2 : Gain  Gain=Xcomp
  Gain3 : Gain  Gain=-1
  Gain4 : Gain  Gain=-1
  Gain5 : Gain  Gain=1/Rsw*traprule
  Gain6 : Gain  Gain=traprule
  Gain7 : Gain  Gain=-1/Rsw
  PS-Simulink Converter2 : nesl_utility/PS-Simulink Converter  PhysicalDomain=network_engine_domain  SubClassName=ps_output  LeftPortType=input  RightPortType=output  PseudoPeriodic=off  Frequencies=[]  VectorFormat=inherit  Unit=inherit  AffineConversion=off
  Relational Operator1 : RelationalOperator  Operator=~=  OutDataTypeStr=boolean  RndMeth=Simplest  InputSameDT=off
  Resistor : fl_lib/Electrical/Electrical Elements/Resistor  R=Rsw Ohm  i_specify=off  i_priority=None  i=0 A  i_nominal_specify=off  i_nominal_value=1  i_nominal_unit=A  v_specify=off  v_priority=None  v=0 V  v_nominal_specify=off  v_nominal_value=1  v_nominal_unit=V
  Simulink-PS Converter1 : nesl_utility/Simulink-PS Converter  PhysicalDomain=network_engine_domain  SubClassName=ps_input  LeftPortType=input  RightPortType=output  PseudoPeriodic=off  Frequencies=[]  NoiseDistribution=none  NoiseParameters=[]  Unit=1  AffineConversion=off  FilteringAndDerivatives=provide  SimscapeFilterOrder=1  InputFilterTimeConstant=0.001  UdotUserProvided=0
  Switch : Switch  Criteria=u2 > Threshold  Threshold=0.5  SaturateOnIntegerOverflow=off  InputSameDT=off
  Switch4 : Switch  Criteria=u2 > Threshold  Threshold=0.5  SaturateOnIntegerOverflow=off  InputSameDT=off
  Switch5 : Switch  Criteria=u2 ~= 0  Threshold=0.5  SaturateOnIntegerOverflow=off  InputSameDT=off
  Unit Delay1 : UnitDelay  SampleTime=-1
  Unit Delay2 : UnitDelay  SampleTime=Ts
  Unit Delay6 : UnitDelay  SampleTime=Ts
  VS1 : fl_lib/Electrical/Electrical Sensors/Voltage Sensor
  init_in : Constant
  init_out : Terminator
  +V : PMIOPort  Side=Left
  -V : PMIOPort  Port=2  Side=Right
  v : Outport
  i : Outport  Port=2
  wires:
  Add4/1 -> [Vsw], v/1
  Add3/1 -> Simulink-PS Converter1/1
  Gain7/1 -> Add3/2
  [Ihist] -> Add3/1
  Vf/1 -> Gain7/1, Add4/2
  Gain6/1 -> Add2/2
  Add2/1 -> Switch/3
  Gain5/1 -> Add1/2
  [Vsw] -> Gain5/1
  Add1/1 -> Switch/1
  Gain4/1 -> i/1
  Switch5/1 -> [Ihist]
  init_in/1 -> Unit Delay2/1
  Relational Operator1/1 -> Gain2/1
  gate/1 -> Switch/2, Relational Operator1/2, Unit Delay6/1, Switch4/2
  Unit Delay6/1 -> Relational Operator1/1
  Gain2/1 -> Switch5/2
  Gain3/1 -> Switch4/1
  Switch4/1 -> init_out/1
  Unit Delay1/1 -> Switch5/3
  Gain1/1 -> Add/2, Add2/1
  [Ihist] -> Add/1
  PS-Simulink Converter2/1 -> Add4/1
  [Vsw] -> Gain1/1
  Switch/1 -> Unit Delay1/1
  Add/1 -> Gain4/1, Add1/1, Gain6/1
  [Ihist] -> Switch4/3, Gain3/1
  Unit Delay2/1 -> Switch5/1
  connections:
  Resistor/RConn1 -- CCS1/LConn1 -- VS1/RConn2 -- -V/RConn1
  PS-Simulink Converter2/LConn1 -- VS1/RConn1
  CCS1/RConn1 -- Simulink-PS Converter1/RConn1
  Resistor/LConn1 -- VS1/LConn1 -- +V/RConn1 -- CCS1/RConn2

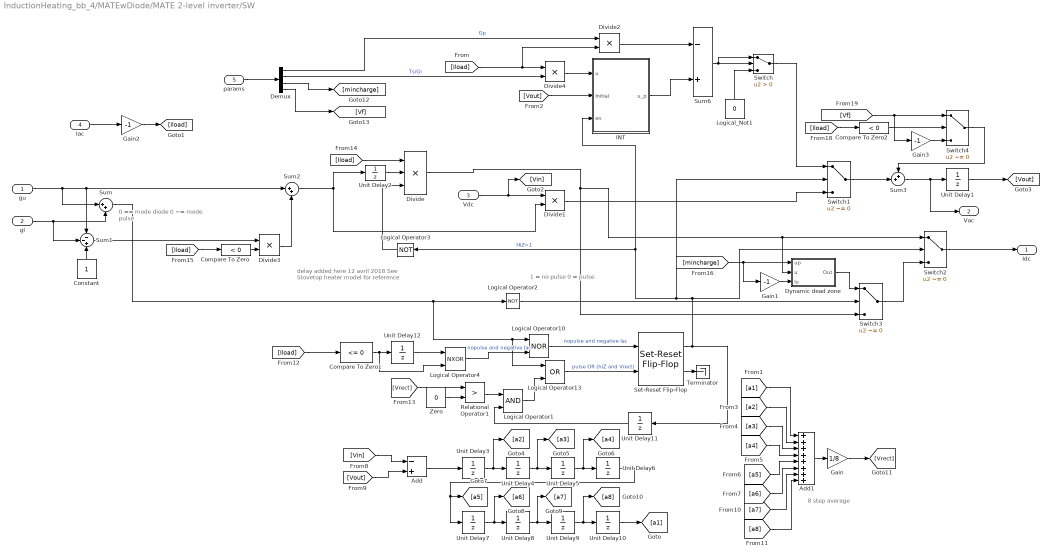
== system InductionHeating_bb_4/MATEwDiode/MATE 2-level inverter/SW ==
  note: 8 step average
  note: 1 = no pulse
      | 0 = pulse
  note: 0 == mode diode
      | 0 ~= mode pulse
  note: delay added here 12 avril 2018
      | See Stovetop heater model for reference
  gu : Inport
  gl : Inport  Port=2
  Vdc : Inport  Port=3
  Iac : Inport  Port=4
  params : Inport  Port=5
  Add : Sum  Inputs=-+
  Add1 : Sum  Inputs=8
  Compare To Zero : simulink/Logic and Bit Operations/Compare To Zero  relop=<  OutDataTypeStr=uint8
  Compare To Zero1 : simulink/Logic and Bit Operations/Compare To Zero  relop=<=  OutDataTypeStr=uint8
  Compare To Zero2 : simulink/Logic and Bit Operations/Compare To Zero  relop=<  OutDataTypeStr=uint8
  Constant : Constant
  Demux : Demux
  Divide : Product  Inputs=3
  Divide{1..4} (4 alike) : Product
  Dynamic dead zone : Subsystem
  Gain : Gain  Gain=1/8
  Gain1 : Gain  Gain=-1
  Gain2 : Gain  Gain=-1
  Gain3 : Gain  Gain=-1
  INT : Subsystem
  Logical Operator1 : Logic  AllPortsSameDT=off  OutDataTypeStr=boolean
  Logical Operator10 : Logic  Operator=NOR  AllPortsSameDT=off  OutDataTypeStr=boolean
  Logical Operator13 : Logic  Operator=OR  AllPortsSameDT=off  OutDataTypeStr=boolean
  Logical Operator2 : Logic  Operator=NOT  AllPortsSameDT=off  OutDataTypeStr=boolean
  Logical Operator3 : Logic  Operator=NOT  AllPortsSameDT=off  OutDataTypeStr=boolean
  Logical Operator4 : Logic  Operator=NXOR  AllPortsSameDT=off  OutDataTypeStr=boolean
  Logical_Not1 : Constant  Value=0  SampleTime=-1
  Relational Operator1 : RelationalOperator  Operator=>  OutDataTypeStr=boolean  InputSameDT=off
  Set-Reset Flip-Flop : eeGeneralControl/Set-Reset Flip-Flop  LabelModeActiveChoice=Discrete  UndefState=Set  Q0=0  Ts=Ts
  Sum : Sum  Inputs=|++
  Sum1 : Sum  Inputs=--+
  Sum2 : Sum  Inputs=|++
  Sum3 : Sum  Inputs=++|
  Sum6 : Sum  Inputs=-+  InputSameDT=on  SaturateOnIntegerOverflow=on  SampleTime=Ts  OutDataTypeStr=Inherit: Same as first input
  Switch : Switch  Criteria=u2 > Threshold  SaturateOnIntegerOverflow=off  InputSameDT=off
  Switch1 : Switch  Criteria=u2 ~= 0  SaturateOnIntegerOverflow=off  InputSameDT=off
  Switch2 : Switch  Criteria=u2 ~= 0  Threshold=0.5  SaturateOnIntegerOverflow=off  InputSameDT=off
  Switch3 : Switch  Criteria=u2 ~= 0  Threshold=0.5  SaturateOnIntegerOverflow=off  InputSameDT=off
  Switch4 : Switch  Criteria=u2 ~= 0  Threshold=0.5  SaturateOnIntegerOverflow=off  InputSameDT=off
  Terminator : Terminator
  Unit Delay{1..12} (12 alike) : UnitDelay  SampleTime=Ts
  Zero : Constant  Value=0  OutDataTypeStr=Inherit: Inherit via back propagation
  Idc : Outport  VectorParamsAs1DForOutWhenUnconnected=off
  Vac : Outport  Port=2  VectorParamsAs1DForOutWhenUnconnected=off
  wires:
  Logical Operator4/1 -> Logical Operator10/2  "nopulse and negative Iac"
  Unit Delay12/1 -> Logical Operator4/1
  Unit Delay10/1 -> [a1]
  Unit Delay2/1 -> Divide/2
  Switch4/1 -> Sum3/1
  Gain3/1 -> Switch4/3
  [Vf] -> Switch4/1, Gain3/1
  Compare To Zero2/1 -> Switch4/2
  Sum3/1 -> Vac/1, Unit Delay1/1
  [Iload] -> Compare To Zero2/1
  Demux/4 -> [Vf]
  params/1 -> Demux/1
  Gain1/1 -> Dynamic dead zone/3(lo)
  [mincharge] -> Gain1/1, Dynamic dead zone/1(up)
  Demux/3 -> [mincharge]
  Demux/2 -> Divide4/2  "Ts/Gi"
  Divide4/1 -> INT/1(u)
  Divide2/1 -> Sum6/1
  Demux/1 -> Divide2/1  "Gp"
  Gain2/1 -> [Iload]
  Sum1/1 -> Divide3/1
  Compare To Zero/1 -> Divide3/2
  [Iload] -> Compare To Zero/1
  [Iload] -> Divide/1
  [Iload] -> Divide2/2, Divide4/1
  Logical Operator1/1 -> Logical Operator13/2
  Logical Operator13/1 -> Set-Reset Flip-Flop/2  "pulse OR (hiZ and Vrect)"
  Unit Delay11/1 -> Logical Operator1/2
  Relational Operator1/1 -> Logical Operator1/1
  Zero/1 -> Relational Operator1/2
  [Vrect] -> Relational Operator1/1
  INT/1(u_p) -> Sum6/2
  Compare To Zero1/1 -> Unit Delay12/1, Logical Operator4/2
  [Iload] -> Compare To Zero1/1
  Gain/1 -> [Vrect]
  Add1/1 -> Gain/1
  [a1] -> Add1/1
  [a8] -> Add1/8
  [a2] -> Add1/2
  [a7] -> Add1/7
  [a6] -> Add1/6
  [a3] -> Add1/3
  [a5] -> Add1/5
  [a4] -> Add1/4
  Unit Delay9/1 -> Unit Delay10/1, [a8]
  Unit Delay8/1 -> Unit Delay9/1, [a7]
  Unit Delay7/1 -> Unit Delay8/1, [a6]
  Unit Delay6/1 -> Unit Delay7/1, [a5]
  Unit Delay5/1 -> Unit Delay6/1, [a4]
  Unit Delay4/1 -> Unit Delay5/1, [a3]
  Unit Delay3/1 -> Unit Delay4/1, [a2]
  Add/1 -> Unit Delay3/1
  [Vout] -> Add/2
  [Vin] -> Add/1
  [Vout] -> INT/2(Initial)
  Logical Operator10/1 -> Set-Reset Flip-Flop/1  "nopulse and negative Iac"
  Unit Delay1/1 -> [Vout]
  Switch3/1 -> Switch2/3
  Dynamic dead zone/1(Out) -> Switch3/1
  Divide/1 -> Switch2/1, Dynamic dead zone/2(u), Switch3/3
  Switch2/1 -> Idc/1
  Switch/1 -> Switch1/1
  Divide1/1 -> Switch1/3
  Sum2/1 -> Unit Delay2/1, Divide1/2
  gu/1 -> Sum1/1, Sum2/1, Sum/1
  Sum/1 -> Logical Operator2/1, Logical Operator10/1, Logical Operator13/1
  Vdc/1 -> [Vin], Divide1/1
  Logical Operator2/1 -> Switch3/2
  Logical Operator3/1 -> Divide/3
  gl/1 -> Sum/2, Sum1/2
  Constant/1 -> Sum1/3
  Divide3/1 -> Sum2/2
  Switch1/1 -> Sum3/2
  Sum6/1 -> Switch/2, Switch/1
  Logical_Not1/1 -> Switch/3
  Set-Reset Flip-Flop/1 -> Unit Delay11/1, Switch2/2, Switch1/2, INT/3(en), Logical Operator3/1  "HiZ=1"
  Iac/1 -> Gain2/1
  Set-Reset Flip-Flop/2 -> Terminator/1

== system InductionHeating_bb_4/MATEwDiode/RL1/RC.1 ==
  RLC : Inport
  typ : Inport  Port=2
  Bus Creator : BusCreator  Inputs=2
  Demux : Demux  Outputs=2
  Divide : Product  Inputs=*/
  Divide1 : Product  Inputs=/
  Divide3 : Product
  Divide4 : Product  Inputs=/
  Divide5 : Product  Inputs=/
  Gain : Gain  Gain=-Ts
  Gain1 : Gain  Gain=Ts/2
  Gain2 : Gain  Gain=Ts/2
  Gain3 : Gain  Gain=-Ts
  Switch : Switch  Criteria=u2 > Threshold  SaturateOnIntegerOverflow=off  InputSameDT=off
  Switch1 : Switch  Criteria=u2 > Threshold  SaturateOnIntegerOverflow=off  InputSameDT=off
  AhB : Outport
  wires:
  Divide5/1 -> Divide3/1
  Demux/2 -> Divide4/1, Divide/2, Divide1/1
  Divide/1 -> Gain/1
  Divide1/1 -> Gain1/1
  Demux/1 -> Divide/1, Divide5/1
  Bus Creator/1 -> AhB/1
  RLC/1 -> Demux/1
  Divide4/1 -> Gain2/1, Divide3/2
  Divide3/1 -> Gain3/1
  Switch/1 -> Bus Creator/1  "Ah"
  Switch1/1 -> Bus Creator/2  "Bh/2"
  typ/1 -> Switch1/2, Switch/2
  Gain/1 -> Switch/3  "Ah"
  Gain1/1 -> Switch1/3  "Bh/2"
  Gain3/1 -> Switch/1  "Ah"
  Gain2/1 -> Switch1/1  "Bh/2"

== system InductionHeating_bb_4/MATEwDiode/RL1/Rsw ==
  Variable Resistor : fl_lib/Electrical/Electrical Elements/Variable Resistor  Rmin=1e-8 Ohm  thermalEnable=false  thermal_mass=1 J/K  i_specify=off  i_priority=None  i=0 A  i_nominal_specify=off  i_nominal_value=1  i_nominal_unit=A  v_specify=off  v_priority=None  v=0 V  v_nominal_specify=off  v_nominal_value=1  v_nominal_unit=V  T_specify=off  T_priority=None  T=300 K  T_nominal_specify=off  T_nominal_value=1  T_nominal_unit=K
  + : PMIOPort  Side=Left
  R : PMIOPort  Port=2  Side=Left
  - : PMIOPort  Port=3  Side=Right
  connections:
  R/RConn1 -- Variable Resistor/LConn1
  Variable Resistor/LConn2 -- +/RConn1
  Variable Resistor/RConn1 -- -/RConn1

== system InductionHeating_bb_4/MATEwDiode/RL1/state_init ==
  in : Inport
  g : Inport  Port=2
  Gain18 : Gain
  Relational Operator1 : RelationalOperator  Operator=~=  OutDataTypeStr=boolean  RndMeth=Simplest  InputSameDT=off
  Switch16 : Switch  Criteria=u2 ~= 0  Threshold=0.5  SaturateOnIntegerOverflow=off  InputSameDT=off
  Unit Delay6 : UnitDelay  SampleTime=-1
  Unit Delay7 : UnitDelay  SampleTime=Ts
  Unit Delay8 : UnitDelay  SampleTime=Ts
  init_in : Constant  Value=0
  out : Outport
  wires:
  g/1 -> Relational Operator1/2, Unit Delay8/1
  Switch16/1 -> out/1
  in/1 -> Unit Delay6/1
  Unit Delay7/1 -> Switch16/1
  Gain18/1 -> Switch16/2
  init_in/1 -> Unit Delay7/1
  Unit Delay6/1 -> Switch16/3
  Relational Operator1/1 -> Gain18/1
  Unit Delay8/1 -> Relational Operator1/1

== system InductionHeating_bb_4/soc16/DynamicMultMAT/add1 ==
  E : Inport
  In1 : Inport  Port=2
  In2 : Inport  Port=3
  In4 : Inport  Port=4
  In5 : Inport  Port=5
  In7 : Inport  Port=6
  In8 : Inport  Port=7
  In10 : Inport  Port=8
  In11 : Inport  Port=9
  Add{3..6} (4 alike) : Sum
  Unit Delay Enabled Synchronous{1..3,22} (4 alike) : hdlsllib/Discrete/Unit Delay Enabled Synchronous  InitialCondition=0.0  SampleTime=-1
  y : Outport
  y1 : Outport  Port=2
  y2 : Outport  Port=3
  y3 : Outport  Port=4
  wires:
  Add4/1 -> Unit Delay Enabled Synchronous1/1
  In1/1 -> Add3/1
  In5/1 -> Add4/2
  Add6/1 -> Unit Delay Enabled Synchronous3/1
  Add3/1 -> Unit Delay Enabled Synchronous22/1
  Add5/1 -> Unit Delay Enabled Synchronous2/1
  Unit Delay Enabled Synchronous1/1 -> y1/1
  Unit Delay Enabled Synchronous3/1 -> y3/1
  E/1 -> Unit Delay Enabled Synchronous3/2, Unit Delay Enabled Synchronous2/2, Unit Delay Enabled Synchronous1/2, Unit Delay Enabled Synchronous22/2
  In4/1 -> Add4/1
  In8/1 -> Add5/2
  In2/1 -> Add3/2
  In10/1 -> Add6/1
  Unit Delay Enabled Synchronous2/1 -> y2/1
  Unit Delay Enabled Synchronous22/1 -> y/1
  In7/1 -> Add5/1
  In11/1 -> Add6/2
